simulink model "ActiveSuspensionv2"  (R2026b)
settings: Solver=ode3  StartTime=0  StopTime=5  FixedStep=0.001
values from neighbouring files (symbols this model uses):
  A = %.12g B=    [ejecutar_pso_30.m]    (also in parameters.m = 10)
  B = 10    [parameters.m]
  B1 = 0    [parameters.m]
  B2 = 1500    [parameters.m]
  C = 4444    [parameters.m]
  K1 = 160000    [parameters.m]
  K2 = 16000    [parameters.m]
  M1 = 50    [parameters.m]
  M2 = 250    [parameters.m]
libraries: simulink x2, fuzblock x1
settings Model: SimulationMode=accelerator  Creator=bug  LastModifiedBy=Elvis
settings DataIOCC: ReturnWorkspaceOutputs=off
settings DebuggingCC: MergeDetectMultiDrivingBlocksExec=none  UnderspecifiedInitializationDetection=Classic
settings ModelReferenceCC: PropagateSignalLabelsOutOfModel=off

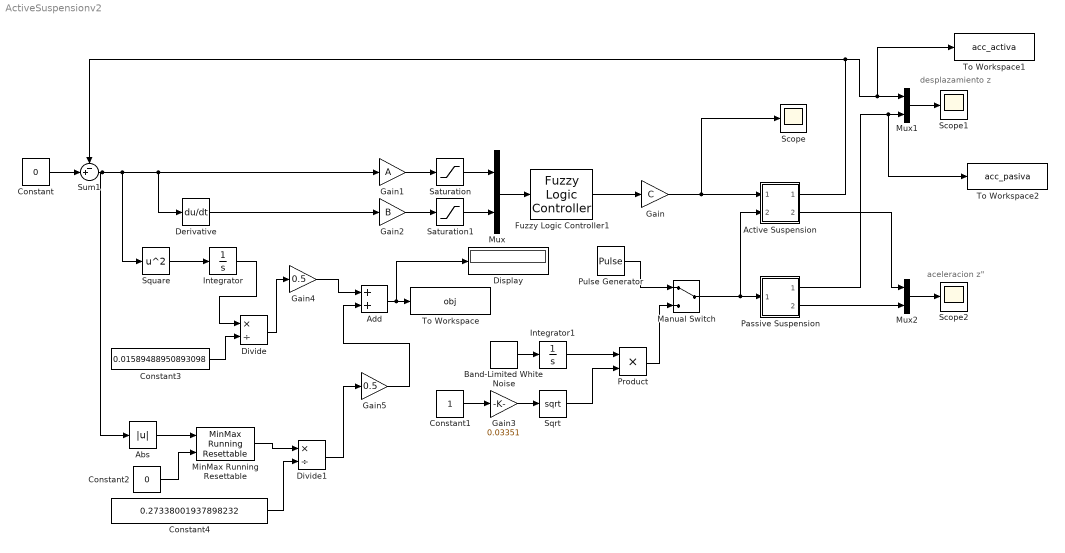
== system ActiveSuspensionv2 ==
  note: desplazamiento z
  note: aceleracion z"
  Abs : Abs  SaturateOnIntegerOverflow=off
  Active Suspension : Subsystem
  Add : Sum
  Band-Limited White Noise : simulink/Sources/Band-Limited White Noise  Cov=[0.1]  Ts=0.001  seed=[23341]
  Constant : Constant  Value=0
  Constant1 : Constant
  Constant2 : Constant  Value=0
  Constant3 : Constant  Value=0.01589488950893098
  Constant4 : Constant  Value=0.27338001937898232
  Derivative : Derivative
  Display : Display
  Divide : Product  Inputs=*/
  Divide1 : Product  Inputs=*/
  Fuzzy Logic Controller1 : fuzblock/Fuzzy Logic  Controller  FIS='suspension.fis'  OutputSampleNumber=101  DataType=double  UseLookupTable=off  NumBreakpoints=10  FuzzifiedInputs=off  RuleFiringStrengths=off  RuleOutputs=off  AggregatedOutputs=off  SimulateUsing=Interpreted execution  OutOfRangeInputValueMessage=warning  NoRuleFiredMessage=warning  EmptyOutputFuzzySetMessage=warning
  Gain : Gain  Gain=C  SaturateOnIntegerOverflow=on  OutDataTypeStr=Inherit: Same as input  ParamDataTypeStr=Inherit: Same as input
  Gain1 : Gain  Gain=A  SaturateOnIntegerOverflow=on  OutDataTypeStr=Inherit: Same as input  ParamDataTypeStr=Inherit: Same as input
  Gain2 : Gain  Gain=B  SaturateOnIntegerOverflow=on  OutDataTypeStr=Inherit: Same as input  ParamDataTypeStr=Inherit: Same as input
  Gain3 : Gain  Gain=0.03351  SaturateOnIntegerOverflow=on  OutDataTypeStr=Inherit: Same as input  ParamDataTypeStr=Inherit: Same as input
  Gain4 : Gain  Gain=0.5
  Gain5 : Gain  Gain=0.5
  Integrator : Integrator
  Integrator1 : Integrator
  Manual Switch : ManualSwitch
  MinMax Running Resettable : simulink/Math Operations/MinMax Running Resettable  Function=max  vinit=0.0
  Mux : Mux  Inputs=2
  Mux1 : Mux  Inputs=2
  Mux2 : Mux  Inputs=2
  Passive Suspension : Subsystem
  Product : Product
  Pulse Generator : DiscretePulseGenerator  PulseType=Time based  Amplitude=0.2  Period=10  PulseWidth=2.5  PhaseDelay=1
  Saturation : Saturate  UpperLimit=1  LowerLimit=-1
  Saturation1 : Saturate  UpperLimit=1  LowerLimit=-1
  Scope : Scope
      settings: ActiveDisplayYMinimum=-4883.9572  ActiveDisplayYMaximum=4882.5596  DataLoggingSaveFormat=Array
  Scope1 : Scope
      settings: ActiveDisplayYMinimum=-0.14334  ActiveDisplayYMaximum=0.31968  DataLoggingSaveFormat=Array
  Scope2 : Scope
      settings: ActiveDisplayYMinimum=-69.26626  ActiveDisplayYMaximum=62.9571  DataLoggingSaveFormat=Array
  Sqrt : Sqrt
  Square : Math  Operator=square
  Sum1 : Sum  Inputs=-+|
  To Workspace : ToWorkspace  VariableName=obj  SaveFormat=Timeseries  SampleTime=-1
  To Workspace1 : ToWorkspace  VariableName=acc_activa  SaveFormat=Timeseries  SampleTime=-1
  To Workspace2 : ToWorkspace  VariableName=acc_pasiva  SaveFormat=Timeseries  SampleTime=-1
  wires:
  Saturation/1 -> Mux/1
  Saturation1/1 -> Mux/2
  Gain1/1 -> Saturation/1
  Gain2/1 -> Saturation1/1
  Sum1/1 -> Square/1, Derivative/1, Gain1/1, Abs/1
  Derivative/1 -> Gain2/1
  Manual Switch/1 -> Active Suspension/2(In2), Passive Suspension/1(In2)
  Pulse Generator/1 -> Manual Switch/1
  Mux1/1 -> Scope1/1
  Constant/1 -> Sum1/2
  Mux/1 -> Fuzzy Logic Controller1/1
  Fuzzy Logic Controller1/1 -> Gain/1
  Gain/1 -> Active Suspension/1(In1), Scope/1
  Mux2/1 -> Scope2/1
  Active Suspension/2(Out2) -> Mux2/1
  Passive Suspension/2(Out2) -> Mux2/2
  Band-Limited White Noise/1 -> Integrator1/1
  Constant1/1 -> Gain3/1
  Gain3/1 -> Sqrt/1
  Sqrt/1 -> Product/2
  Integrator1/1 -> Product/1
  Product/1 -> Manual Switch/2
  Passive Suspension/1(Out1) -> To Workspace2/1, Mux1/2
  Active Suspension/1(Out1) -> To Workspace1/1, Mux1/1, Sum1/1
  Constant2/1 -> MinMax Running Resettable/2
  Abs/1 -> MinMax Running Resettable/1
  Square/1 -> Integrator/1
  Gain4/1 -> Add/1
  Gain5/1 -> Add/2
  Add/1 -> Display/1, To Workspace/1
  MinMax Running Resettable/1 -> Divide1/1
  Divide1/1 -> Gain5/1
  Integrator/1 -> Divide/1
  Divide/1 -> Gain4/1
  Constant4/1 -> Divide1/2
  Constant3/1 -> Divide/2

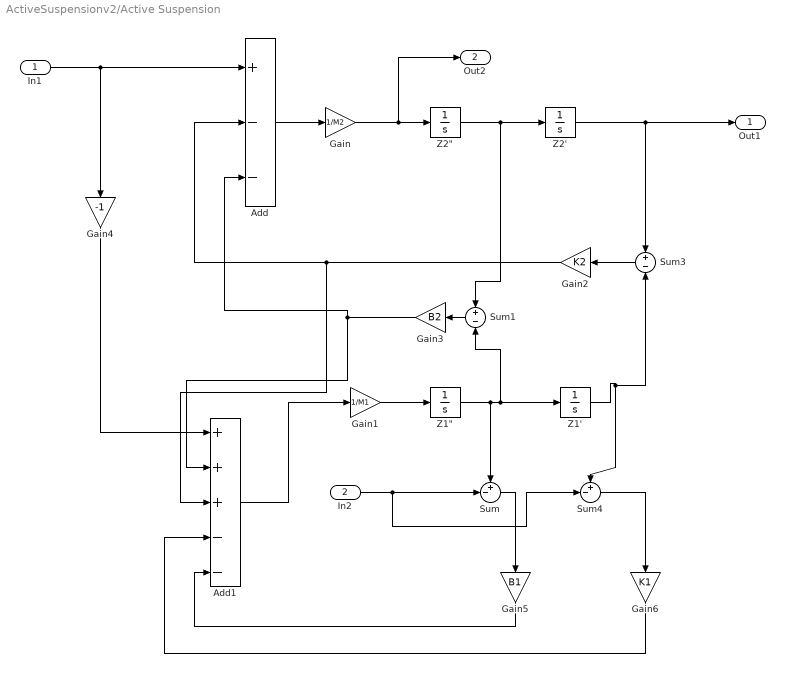
== system ActiveSuspensionv2/Active Suspension ==
  In1 : Inport
  In2 : Inport  Port=2
  Add : Sum  Inputs=+--  InputSameDT=on  SaturateOnIntegerOverflow=on  OutDataTypeStr=Inherit: Same as first input
  Add1 : Sum  Inputs=+++--  InputSameDT=on  SaturateOnIntegerOverflow=on  OutDataTypeStr=Inherit: Same as first input
  Gain : Gain  Gain=1/M2  SaturateOnIntegerOverflow=on  OutDataTypeStr=Inherit: Same as input  ParamDataTypeStr=Inherit: Same as input
  Gain1 : Gain  Gain=1/M1  SaturateOnIntegerOverflow=on  OutDataTypeStr=Inherit: Same as input  ParamDataTypeStr=Inherit: Same as input
  Gain2 : Gain  Gain=K2  SaturateOnIntegerOverflow=on  OutDataTypeStr=Inherit: Same as input  ParamDataTypeStr=Inherit: Same as input
  Gain3 : Gain  Gain=B2  SaturateOnIntegerOverflow=on  OutDataTypeStr=Inherit: Same as input  ParamDataTypeStr=Inherit: Same as input
  Gain4 : Gain  Gain=-1  SaturateOnIntegerOverflow=on  OutDataTypeStr=Inherit: Same as input  ParamDataTypeStr=Inherit: Same as input
  Gain5 : Gain  Gain=B1  SaturateOnIntegerOverflow=on  OutDataTypeStr=Inherit: Same as input  ParamDataTypeStr=Inherit: Same as input
  Gain6 : Gain  Gain=K1  SaturateOnIntegerOverflow=on  OutDataTypeStr=Inherit: Same as input  ParamDataTypeStr=Inherit: Same as input
  Sum : Sum  Inputs=+-|
  Sum1 : Sum  Inputs=+-
  Sum3 : Sum  Inputs=+-
  Sum4 : Sum  Inputs=+-|
  "Z1\"" : Integrator
  Z1' : Integrator
  "Z2\"" : Integrator
  Z2' : Integrator
  Out1 : Outport
  Out2 : Outport  Port=2
  wires:
  Gain3/1 -> Add/3, Add1/2
  Gain2/1 -> Add1/3, Add/2
  "Z2\""/1 -> Sum1/1, Z2'/1
  In1/1 -> Add/1, Gain4/1
  Gain1/1 -> "Z1\""/1
  Gain/1 -> Out2/1, "Z2\""/1
  Add/1 -> Gain/1
  Add1/1 -> Gain1/1
  Z2'/1 -> Sum3/1, Out1/1
  Z1'/1 -> Sum3/2, Sum4/1
  In2/1 -> Sum4/2, Sum/2
  Gain4/1 -> Add1/1
  Sum3/1 -> Gain2/1
  Gain5/1 -> Add1/5
  Gain6/1 -> Add1/4
  Sum/1 -> Gain5/1
  "Z1\""/1 -> Sum/1, Sum1/2, Z1'/1
  Sum4/1 -> Gain6/1
  Sum1/1 -> Gain3/1

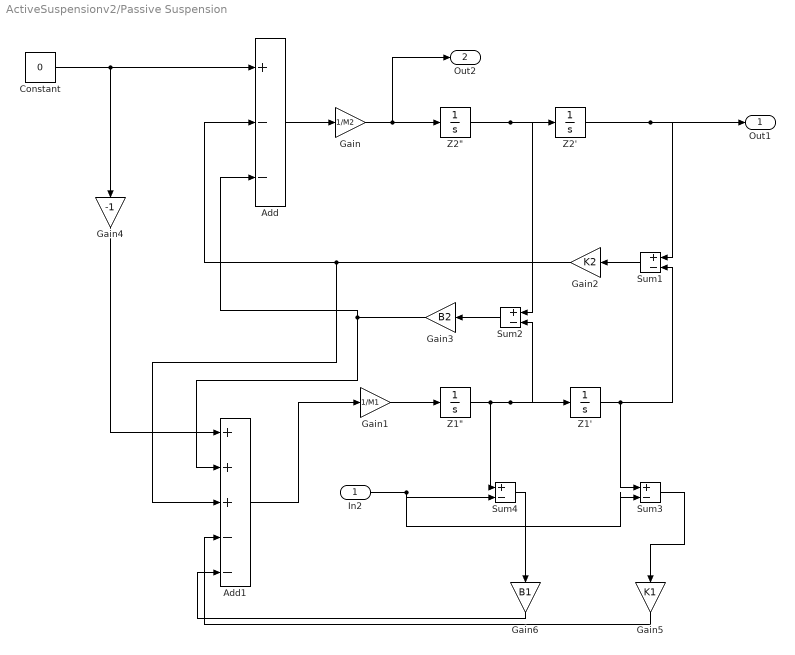
== system ActiveSuspensionv2/Passive Suspension ==
  In2 : Inport
  Add : Sum  Inputs=+--  InputSameDT=on  SaturateOnIntegerOverflow=on  OutDataTypeStr=Inherit: Same as first input
  Add1 : Sum  Inputs=+++--  InputSameDT=on  SaturateOnIntegerOverflow=on  OutDataTypeStr=Inherit: Same as first input
  Constant : Constant  Value=0
  Gain : Gain  Gain=1/M2  SaturateOnIntegerOverflow=on  OutDataTypeStr=Inherit: Same as input  ParamDataTypeStr=Inherit: Same as input
  Gain1 : Gain  Gain=1/M1  SaturateOnIntegerOverflow=on  OutDataTypeStr=Inherit: Same as input  ParamDataTypeStr=Inherit: Same as input
  Gain2 : Gain  Gain=K2  SaturateOnIntegerOverflow=on  OutDataTypeStr=Inherit: Same as input  ParamDataTypeStr=Inherit: Same as input
  Gain3 : Gain  Gain=B2  SaturateOnIntegerOverflow=on  OutDataTypeStr=Inherit: Same as input  ParamDataTypeStr=Inherit: Same as input
  Gain4 : Gain  Gain=-1  SaturateOnIntegerOverflow=on  OutDataTypeStr=Inherit: Same as input  ParamDataTypeStr=Inherit: Same as input
  Gain5 : Gain  Gain=K1  SaturateOnIntegerOverflow=on  OutDataTypeStr=Inherit: Same as input  ParamDataTypeStr=Inherit: Same as input
  Gain6 : Gain  Gain=B1  SaturateOnIntegerOverflow=on  OutDataTypeStr=Inherit: Same as input  ParamDataTypeStr=Inherit: Same as input
  Sum1 : Sum  Inputs=+-  InputSameDT=on  SaturateOnIntegerOverflow=on  OutDataTypeStr=Inherit: Same as first input
  Sum2 : Sum  Inputs=+-  InputSameDT=on  SaturateOnIntegerOverflow=on  OutDataTypeStr=Inherit: Same as first input
  Sum3 : Sum  Inputs=+-|  InputSameDT=on  SaturateOnIntegerOverflow=on  OutDataTypeStr=Inherit: Same as first input
  Sum4 : Sum  Inputs=+-|  InputSameDT=on  SaturateOnIntegerOverflow=on  OutDataTypeStr=Inherit: Same as first input
  "Z1\"" : Integrator
  Z1' : Integrator
  "Z2\"" : Integrator
  Z2' : Integrator
  Out1 : Outport
  Out2 : Outport  Port=2
  wires:
  Gain3/1 -> Add/3, Add1/2
  Gain2/1 -> Add1/3, Add/2
  "Z2\""/1 -> Sum2/1, Z2'/1
  Sum3/1 -> Gain5/1
  Constant/1 -> Add/1, Gain4/1
  Gain1/1 -> "Z1\""/1
  "Z1\""/1 -> Sum4/1, Sum2/2, Z1'/1
  Gain/1 -> Out2/1, "Z2\""/1
  Add/1 -> Gain/1
  Add1/1 -> Gain1/1
  Sum2/1 -> Gain3/1
  Z2'/1 -> Out1/1, Sum1/1
  Sum4/1 -> Gain6/1
  Z1'/1 -> Sum3/1, Sum1/2
  In2/1 -> Sum4/2, Sum3/2
  Gain4/1 -> Add1/1
  Sum1/1 -> Gain2/1
  Gain5/1 -> Add1/4
  Gain6/1 -> Add1/5
